simulink model "Bench_William"  (R2026b)
settings: Solver=ode1  StopTime=T_end  FixedStep=Ts
values from neighbouring files (symbols this model uses):
  du_min = -30    [Bench_run_William.m]
  Ts = 1e-3    (= 0.001)    [Bench_run_William.m]
undefined symbols (not defined in the file or in its folder): ISCS_Ad, ISCS_Bd, ISCS_Cd, ISCS_Dd, ISCS_Tu, ISCS_Ty
settings Model: Creator=williamvandevoir  LastModifiedBy=williamvandevoir

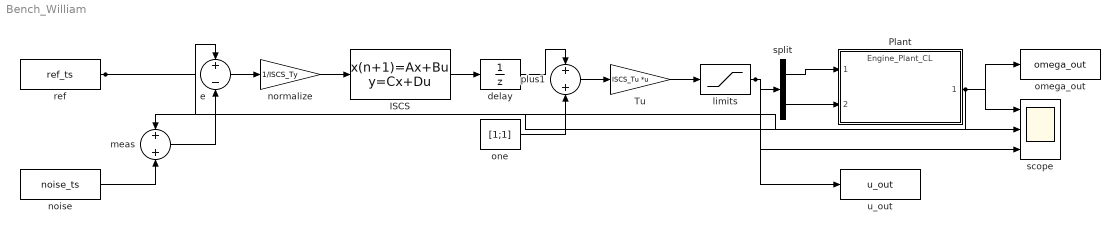
== system Bench_William ==
  ISCS : DiscreteStateSpace  A=ISCS_Ad  B=ISCS_Bd  C=ISCS_Cd  D=ISCS_Dd  InitialCondition=zeros(12,1)  SampleTime=Ts
  Plant : ModelReference  ModelNameDialog=Engine_Plant_CL  SimulationMode=Normal  ModelReferenceVersion=1.23
  Tu : Gain  Gain=ISCS_Tu  Multiplication=Matrix(K*u)
  delay : UnitDelay  InitialCondition=zeros(2,1)  SampleTime=Ts
  e : Sum  Inputs=+-
  limits : Saturate  UpperLimit=[100; 0]  LowerLimit=[0; du_min]
  meas : Sum
  noise : FromWorkspace  VariableName=noise_ts  Interpolate=off  OutputAfterFinalValue=Holding final value
  normalize : Gain  Gain=1/ISCS_Ty
  omega_out : ToWorkspace  VariableName=omega_out  SaveFormat=Timeseries  SampleTime=-1
  one : Constant  Value=[1;1]
  plus1 : Sum
  ref : FromWorkspace  VariableName=ref_ts  Interpolate=off  OutputAfterFinalValue=Holding final value
  scope : Scope  NumInputPorts=3
  split : Demux  Outputs=2
  u_out : ToWorkspace  VariableName=u_out  SaveFormat=Timeseries  SampleTime=-1
  wires:
  ref/1 -> e/1, scope/2
  Plant/1 -> meas/1, omega_out/1, scope/1
  noise/1 -> meas/2
  meas/1 -> e/2
  e/1 -> normalize/1
  normalize/1 -> ISCS/1
  ISCS/1 -> delay/1
  delay/1 -> plus1/1
  one/1 -> plus1/2
  plus1/1 -> Tu/1
  Tu/1 -> limits/1
  limits/1 -> split/1, u_out/1, scope/3
  split/1 -> Plant/1
  split/2 -> Plant/2
